simulink model "Transformer_Operating_Model"  (R2025b)
settings: Solver=ode23t  StartTime=0.0  StopTime=t_stop  MaxStep=t_step_max  RelTol=solver_reltol
PreLoadFcn:
  | if exist('params_transformer','file')~=2, addpath(fileparts(get_param(bdroot,'FileName'))); end; params_transformer;
InitFcn:
  | if exist('params_transformer','file')~=2, addpath(fileparts(get_param(bdroot,'FileName'))); end; params_transformer;
values from neighbouring files (symbols this model uses):
  dT_double_age = 6    [params_transformer.m]
  dTheta_hr = H_hs * g_r    (= 22.1)    [params_transformer.m]
  I_LV_rated = S_rated/(sqrt(3)*V_LV)    [params_transformer.m]
  k21 = 2    [params_transformer.m]
  P0 = 18e3    (= 18000)    [params_transformer.m]
  P_load_min = 1e-3*S_rated    (= 40000)    [params_transformer.m]
  P_tot_r = P0 + Pk    (= 154000)    [params_transformer.m]
  Pk = ukr_pct/100 * S_rated    (= 136000)    [params_transformer.m]
  R_th_h = 1    [params_transformer.m]
  S_rated = 40e6    (= 40000000)    [params_transformer.m]
  t_event_s = 60    [params_transformer.m]
  t_sample_s = t_sample_h*3600    [params_transformer.m]
  T_zero_C_in_K = 273.15    [params_transformer.m]
  theta_amb_C = 20    [params_transformer.m]    (also in run_step36.m = evalin('base', 'theta_amb_C'))
  theta_ref_age = 98    [params_transformer.m]
  x_oil = 0.8    [params_transformer.m]
  y_wdg = 1.3    [params_transformer.m]
libraries: fl_lib x16, nesl_utility x10, ee_lib x4, simulink x1
Description:
  | Transformer operating model (40 MVA, 110/20 kV): electrical network, losses, thermal network and ageing. Operating context only: no gas value is generated. Parameters: params_transformer.m. Built by build_Transformer_Operating_Model.m (MPhil project, Roadmap Step 33).
settings Model: Creator=Silas Asare  LastModifiedBy=Silas Asare
settings DebuggingCC: SignalInfNanChecking=error  UnconnectedInputMsg=error  UnconnectedOutputMsg=error  UnconnectedLineMsg=error  UniqueDataStoreMsg=error  StrictBusMsg=ErrorOnBusTreatedAsVector

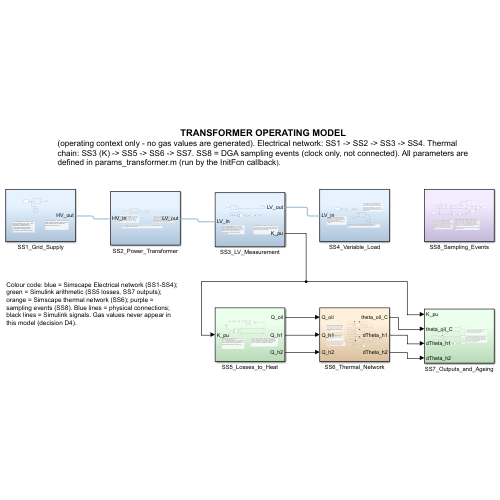
[thumbnail: Simulink's stored preview of the top-level diagram]
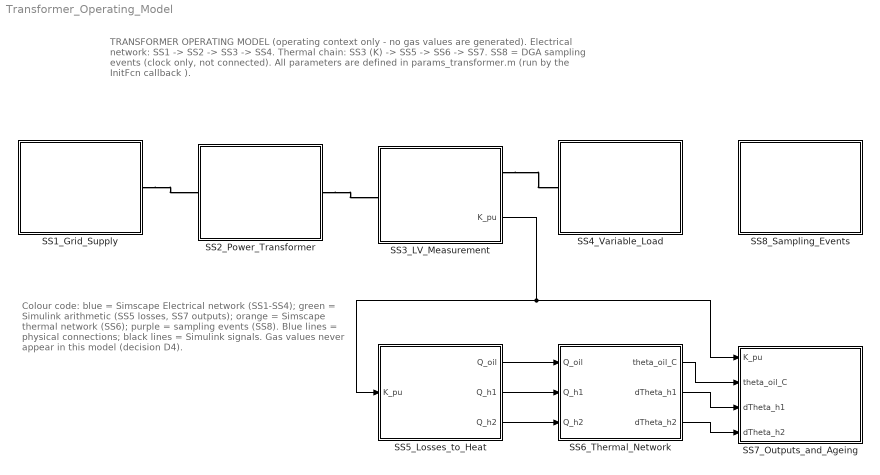
== system Transformer_Operating_Model ==
  note: TRANSFORMER OPERATING MODEL
      | (operating context only - no gas values are generated). Electrical network: SS1 -> SS2 -> SS3 -> SS4. Thermal chain: SS3 (K) -> SS5 -> SS6 -> SS7. SS8 = DGA sampling events (clock only, not connected). All parameters are defined in params_transformer.m (run by the InitFcn callback ).
  note: Colour code: blue = Simscape Electrical network (SS1-SS4); green = Simulink arithmetic (SS5 losses, SS7 outputs); orange = Simscape thermal network (SS6); purple = sampling events (SS8). Blue lines = physical connections; black lines = Simulink signals. Gas values never appear in this model (decision D4).
  SS1_Grid_Supply : Subsystem  Description=Simscape Electrical. Ideal 110 kV, 50 Hz three-phase source (infinite bus). Output HV_out.
  SS2_Power_Transformer : Subsystem  Description=Simscape Electrical. 40 MVA Delta/grounded-Wye transformer with winding resistance, leakage and magnetising branch. HV_in -> LV_out.
  SS3_LV_Measurement : Subsystem  Description=Simscape Electrical sensor + Simulink arithmetic. Measures the LV currents and outputs the load factor K_pu. LV_in -> LV_out, K_pu.
      settings: PortSchema="{\"entries\":[{\"content\":{\"sides\":[{\"content\":{\"connectorIds\":[\"LConn1\"]},\"type\":\"ConnectorPlacement.EquallySpacedRectSide\",\"uuid\":\"625cf4c8-f538-443e-9be6-835b81de7975\"},{\"content\":{\"connectorIds\":[\"RConn1\",\"Out1\"],\"side\":\"RIGHT\"},\"type\":\"ConnectorPlacement.EquallySpacedRectSide\",\"uuid\":\"310d5747-96d2-486e-a648-53e939d57def\"},{\"content\":{\"side\":\"TOP\"},\"type\":\"ConnectorPlacement.EquallySpacedRectSide\",\"uuid\":\"30abf6b0-d060-4f16-93ae-5727792815bb\"}]},\"type\":\"ConnectorPlacement.EquallySpacedConnector\",\"uuid\":\"dfd1b5c5-28ca-4eef-9e4a-4f0f0934eb6f\"}],\"packageUris\":[\"http://schema.mathworks.com/mf0/Connector/R2020b\"],\"version\":\"1.0\"}"
  SS4_Variable_Load : Subsystem  Description=Simscape Electrical + Simulink. Resistive three-phase load, P = K(t)*S_rated, from load_profile. Input LV_in.
  SS5_Losses_to_Heat : Subsystem  Description=Simulink. Heat inputs Q_oil, Q_h1, Q_h2 [W] from K_pu (IEC 60076-7 differential-equation model).
  SS6_Thermal_Network : Subsystem  Description=Simscape Foundation thermal. Three R-C circuits: top oil, hot-spot rise 1 and 2. Own Solver Configuration.
  SS7_Outputs_and_Ageing : Subsystem  Description=Simulink. Hot-spot temperature, relative ageing rate, and logging of K_pu, theta_oil_C, theta_hs_C, ageing_rate_V.
  SS8_Sampling_Events : Subsystem  Description=Simulink. DGA sampling events (Step 37): from the clock and t_sample_s it outputs record_index (row in heldout_record_ids) and sampling_event. Never a gas value; not connected to SS1-SS7.
  wires:
  SS3_LV_Measurement/1(K_pu) -> SS5_Losses_to_Heat/1(K_pu), SS7_Outputs_and_Ageing/1(K_pu)
  SS5_Losses_to_Heat/1(Q_oil) -> SS6_Thermal_Network/1(Q_oil)
  SS6_Thermal_Network/1(theta_oil_C) -> SS7_Outputs_and_Ageing/2(theta_oil_C)
  SS5_Losses_to_Heat/2(Q_h1) -> SS6_Thermal_Network/2(Q_h1)
  SS6_Thermal_Network/2(dTheta_h1) -> SS7_Outputs_and_Ageing/3(dTheta_h1)
  SS5_Losses_to_Heat/3(Q_h2) -> SS6_Thermal_Network/3(Q_h2)
  SS6_Thermal_Network/3(dTheta_h2) -> SS7_Outputs_and_Ageing/4(dTheta_h2)
  connections:
  SS1_Grid_Supply/RConn1 -- SS2_Power_Transformer/LConn1
  SS2_Power_Transformer/RConn1 -- SS3_LV_Measurement/LConn1
  SS3_LV_Measurement/RConn1 -- SS4_Variable_Load/LConn1

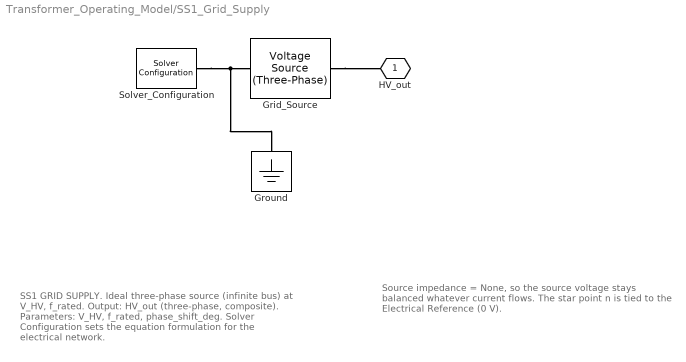
== system Transformer_Operating_Model/SS1_Grid_Supply ==
  note: SS1 GRID SUPPLY. Ideal three-phase source (infinite bus) at V_HV, f_rated. Output: HV_out (three-phase, composite). Parameters: V_HV, f_rated, phase_shift_deg. Solver Configuration sets the equation formulation for the electrical network.
  note: Source impedance = None, so the source voltage stays balanced whatever current flows. The star point n is tied to the Electrical Reference (0 V).
  Grid_Source : ee_lib/Sources/Voltage Source (Three-Phase)  vline_rms=V_HV V  shift=phase_shift_deg deg  freq=f_rated Hz  impedance_option=0  SShortCircuit=1e6 A*V  XR=15  R=0.01 Ohm  L=3.97e-4 H  harmonic_option=0  harmonic_orders=[5, 7, 11, 13]  harmonic_ratios=[.1, .1, .1, .1]  G_parasitic=0 1/Ohm  I_specify=off  I_priority=None  I=[0, 0, 0] A  I_nominal_specify=off  I_nominal_value=1  I_nominal_unit=A
  Ground : fl_lib/Electrical/Electrical Elements/Electrical Reference
  Solver_Configuration : nesl_utility/Solver Configuration  PhysicalDomain=network_engine_domain  SubClassName=solver  LeftPortType=input  RightPortType=generic  Tones=[]  Harmonics=[]  SimulateNoise=off  Profile=off  UseLocalSampling=off  EnableSwitchedLinearOptims=on  FrequencyDomain=off  UseCCode=off  RelTol=0.001  AbsTol=0.001  MinStep=1e-09  ToWorkspace=off  RevertToSquareIcSolve=off  NumHomotopyIterations=100  PhasorMode=off  PhasorModeNumHarmonics=1  ConsistencySolver=NEWTON_XTOL_AFTER_FTOL  IndexReductionMethod=DerivativeReplacement  DoDC=off  ResidualTolerance=1e-09  ConsistencyTolSource=GLOBAL  ConsistencyAbsTol=0.001  ConsistencyRelTol=0.001  ConsistencyTolFactor=0.001  UseLocalSolver=off  LocalSolverChoice=NE_BACKWARD_EULER_ADVANCER  ResolveIndetEquations=on  FunctionEvalNumThread=1  LocalSolverSampleTime=0.001  DoFixedCost=off  MaxNonlinIter=3  MaxModeIter=2  ComputeImpulses=off  ImpulseIterations=2  LinearAlgebra=auto  LinearAlgebraNumThread=0  EquationFormulation=NE_FREQUENCY_TIME_EF  DelaysMemoryBudget=1024  AutomaticFiltering=on  FilteringTimeConstant=0.001  PartitionStorageMethod=AS_NEEDED  PartitionMemoryBudget=1024  PartitionMethod=ROBUST  MultibodyUseLocalSolver=off  MultibodyLocalSolverChoice=ODE1  MultibodyLocalSolverSampleTime=0.001
  HV_out : PMIOPort  Side=Right
  connections:
  Grid_Source/RConn1 -- HV_out/RConn1
  Solver_Configuration/RConn1 -- Ground/LConn1 -- Grid_Source/LConn1

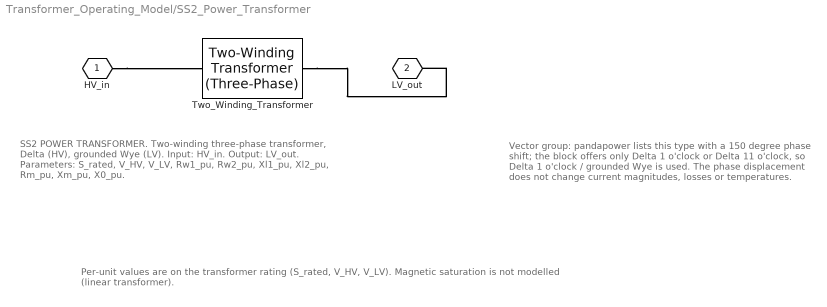
== system Transformer_Operating_Model/SS2_Power_Transformer ==
  note: SS2 POWER TRANSFORMER. Two-winding three-phase transformer, Delta (HV), grounded Wye (LV). Input: HV_in. Output: LV_out. Parameters: S_rated, V_HV, V_LV, Rw1_pu, Rw2_pu, Xl1_pu, Xl2_pu, Rm_pu, Xm_pu, X0_pu.
  note: Vector group: pandapower lists this type with a 150 degree phase shift; the block offers only Delta 1 o'clock or Delta 11 o'clock, so Delta 1 o'clock / grounded Wye is used. The phase displacement does not change current magnitudes, losses or temperatures.
  note: Per-unit values are on the transformer rating (S_rated, V_HV, V_LV). Magnetic saturation is not modelled (linear transformer).
  Two_Winding_Transformer : ee_lib/Passive/Transformers/Two-Winding Transformer (Three-Phase)  SRated=S_rated V*A  FRated=f_rated Hz  Winding1Connection=ee.enum.windingconnection.delta1  VRated1=V_HV V  Winding2Connection=ee.enum.windingconnection.Yg  VRated2=V_LV V  CoreType=ee.enum.coretype.threelimb  pu_Rw1=Rw1_pu  pu_Rw2=Rw2_pu  leakage_reactance_option=ee.enum.transformer_leakage.include  pu_Xl1=Xl1_pu  pu_Xl2=Xl2_pu  magnetizing_resistance_option=ee.enum.transformer_magnetizingResistance.include  pu_Rm=Rm_pu  magnetizing_reactance_option=ee.enum.transformer_magnetizingReactance.include  saturation_option=ee.enum.transformer_saturation.exclude  pu_Xm=Xm_pu  current_data=[0, .002, 1, 2]  magnetic_flux_data=[0, 1.2, 1.5, 1.51]  pu_X0=X0_pu  i1_specify=off  i1_priority=None  i1=[0, 0, 0] A  i1_nominal_specify=off  i1_nominal_value=1  i1_nominal_unit=A  i2_specify=off  i2_priority=None  i2=[0, 0, 0] A  i2_nominal_specify=off  i2_nominal_value=1  i2_nominal_unit=A  phi_specify=off  phi_priority=None  phi=[0, 0, 0]  phi_nominal_specify=off  phi_nominal_value=1  phi_nominal_unit=1  power_dissipated_specify=off  power_dissipated_priority=None  power_dissipated=0 W  power_dissipated_nominal_specify=off  power_dissipated_nominal_value=1  power_dissipated_nominal_unit=W
      settings: InternalSimscapePortConfiguration="{\"Bottom\":[],\"Left\":[{\"id\":\"N1\",\"label\":\"~1\",\"type\":\"foundation.electrical.three_phase\"}],\"Right\":[{\"id\":\"N2\",\"label\":\"~2\",\"type\":\"foundation.electrical.three_phase\"}],\"Top\":[]}"
  HV_in : PMIOPort  Side=Left
  LV_out : PMIOPort  Port=2  Side=Right
  connections:
  HV_in/RConn1 -- Two_Winding_Transformer/LConn1
  Two_Winding_Transformer/RConn1 -- LV_out/RConn1

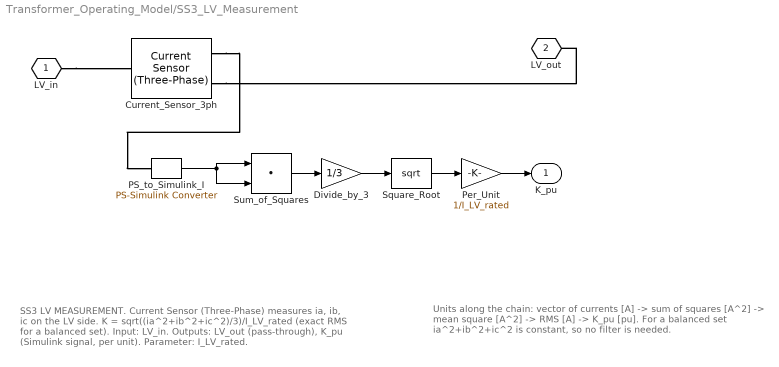
== system Transformer_Operating_Model/SS3_LV_Measurement ==
  note: SS3 LV MEASUREMENT. Current Sensor (Three-Phase) measures ia, ib, ic on the LV side. K = sqrt((ia^2+ib^2+ic^2)/3)/I_LV_rated (exact RMS for a balanced set). Input: LV_in. Outputs: LV_out (pass-through), K_pu (Simulink signal, per unit). Parameter: I_LV_rated.
  note: Units along the chain: vector of currents [A] -> sum of squares [A^2] -> mean square [A^2] -> RMS [A] -> K_pu [pu]. For a balanced set ia^2+ib^2+ic^2 is constant, so no filter is needed.
  Current_Sensor_3ph : ee_lib/Sensors & Transducers/Current Sensor (Three-Phase)
  Divide_by_3 : Gain  Gain=1/3
  PS_to_Simulink_I : nesl_utility/PS-Simulink Converter  PhysicalDomain=network_engine_domain  SubClassName=ps_output  LeftPortType=input  RightPortType=output  PseudoPeriodic=off  Frequencies=[]  VectorFormat=inherit  Unit=A  AffineConversion=off
  Per_Unit : Gain  Gain=1/I_LV_rated
  Square_Root : Sqrt
  Sum_of_Squares : DotProduct  OutDataTypeStr=Inherit: Inherit via internal rule
  LV_in : PMIOPort  Side=Left
  LV_out : PMIOPort  Port=2  Side=Right
  K_pu : Outport
  wires:
  PS_to_Simulink_I/1 -> Sum_of_Squares/1, Sum_of_Squares/2
  Sum_of_Squares/1 -> Divide_by_3/1
  Divide_by_3/1 -> Square_Root/1
  Square_Root/1 -> Per_Unit/1
  Per_Unit/1 -> K_pu/1
  connections:
  LV_in/RConn1 -- Current_Sensor_3ph/LConn1
  Current_Sensor_3ph/RConn2 -- LV_out/RConn1
  Current_Sensor_3ph/RConn1 -- PS_to_Simulink_I/LConn1

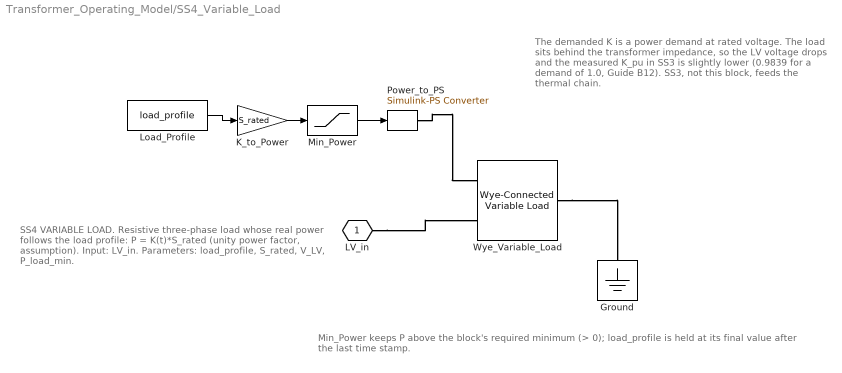
== system Transformer_Operating_Model/SS4_Variable_Load ==
  note: SS4 VARIABLE LOAD. Resistive three-phase load whose real power follows the load profile: P = K(t)*S_rated (unity power factor, assumption). Input: LV_in. Parameters: load_profile, S_rated, V_LV, P_load_min.
  note: The demanded K is a power demand at rated voltage. The load sits behind the transformer impedance, so the LV voltage drops and the measured K_pu in SS3 is slightly lower (0.9839 for a demand of 1.0, Guide B12). SS3, not this block, feeds the thermal chain.
  note: Min_Power keeps P above the block's required minimum (> 0); load_profile is held at its final value after the last time stamp.
  Ground : fl_lib/Electrical/Electrical Elements/Electrical Reference
  K_to_Power : Gain  Gain=S_rated
  Load_Profile : FromWorkspace  VariableName=load_profile  OutputAfterFinalValue=Holding final value
  Min_Power : Saturate  UpperLimit=inf  LowerLimit=P_load_min
  Power_to_PS : nesl_utility/Simulink-PS Converter  PhysicalDomain=network_engine_domain  SubClassName=ps_input  LeftPortType=input  RightPortType=output  PseudoPeriodic=off  Frequencies=[]  NoiseDistribution=none  NoiseParameters=[]  Unit=W  AffineConversion=off  FilteringAndDerivatives=provide  SimscapeFilterOrder=1  InputFilterTimeConstant=0.001  UdotUserProvided=0
  Wye_Variable_Load : ee_lib/Passive/RLC Assemblies/Wye-Connected Variable Load  VRated=V_LV V  Pmin=P_load_min W
      settings: InternalSimscapePortConfiguration="{\"Bottom\":[],\"Left\":[{\"id\":\"P\",\"label\":\"P\",\"type\":\"input\"},{\"id\":\"N\",\"label\":\"~\",\"type\":\"foundation.electrical.three_phase\"}],\"Right\":[{\"id\":\"n\",\"label\":\"n\",\"type\":\"foundation.electrical.electrical\"}],\"Top\":[]}"
  LV_in : PMIOPort  Side=Left
  wires:
  Load_Profile/1 -> K_to_Power/1
  K_to_Power/1 -> Min_Power/1
  Min_Power/1 -> Power_to_PS/1
  connections:
  LV_in/RConn1 -- Wye_Variable_Load/LConn2
  Wye_Variable_Load/RConn1 -- Ground/LConn1
  Power_to_PS/RConn1 -- Wye_Variable_Load/LConn1

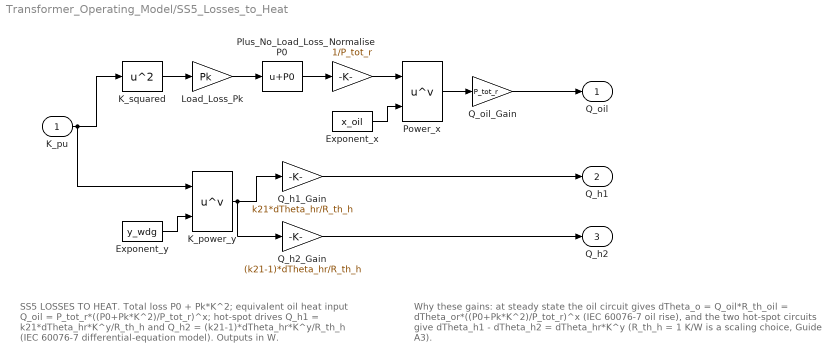
== system Transformer_Operating_Model/SS5_Losses_to_Heat ==
  note: SS5 LOSSES TO HEAT. Total loss P0 + Pk*K^2; equivalent oil heat input Q_oil = P_tot_r*((P0+Pk*K^2)/P_tot_r)^x; hot-spot drives Q_h1 = k21*dTheta_hr*K^y/R_th_h and Q_h2 = (k21-1)*dTheta_hr*K^y/R_th_h (IEC 60076-7 differential-equation model). Outputs in W.
  note: Why these gains: at steady state the oil circuit gives dTheta_o = Q_oil*R_th_oil = dTheta_or*((P0+Pk*K^2)/P_tot_r)^x (IEC 60076-7 oil rise), and the two hot-spot circuits give dTheta_h1 - dTheta_h2 = dTheta_hr*K^y (R_th_h = 1 K/W is a scaling choice, Guide A3).
  K_pu : Inport
  Exponent_x : Constant  Value=x_oil
  Exponent_y : Constant  Value=y_wdg
  K_power_y : Math  Operator=pow
  K_squared : Math  Operator=square
  Load_Loss_Pk : Gain  Gain=Pk
  Normalise : Gain  Gain=1/P_tot_r
  Plus_No_Load_Loss_P0 : Bias  Bias=P0  SaturateOnIntegerOverflow=off
  Power_x : Math  Operator=pow
  Q_h1_Gain : Gain  Gain=k21*dTheta_hr/R_th_h
  Q_h2_Gain : Gain  Gain=(k21-1)*dTheta_hr/R_th_h
  Q_oil_Gain : Gain  Gain=P_tot_r
  Q_oil : Outport
  Q_h1 : Outport  Port=2
  Q_h2 : Outport  Port=3
  wires:
  K_pu/1 -> K_squared/1, K_power_y/1
  K_squared/1 -> Load_Loss_Pk/1
  Load_Loss_Pk/1 -> Plus_No_Load_Loss_P0/1
  Plus_No_Load_Loss_P0/1 -> Normalise/1
  Normalise/1 -> Power_x/1
  Exponent_x/1 -> Power_x/2
  Power_x/1 -> Q_oil_Gain/1
  Q_oil_Gain/1 -> Q_oil/1
  Exponent_y/1 -> K_power_y/2
  K_power_y/1 -> Q_h1_Gain/1, Q_h2_Gain/1
  Q_h1_Gain/1 -> Q_h1/1
  Q_h2_Gain/1 -> Q_h2/1

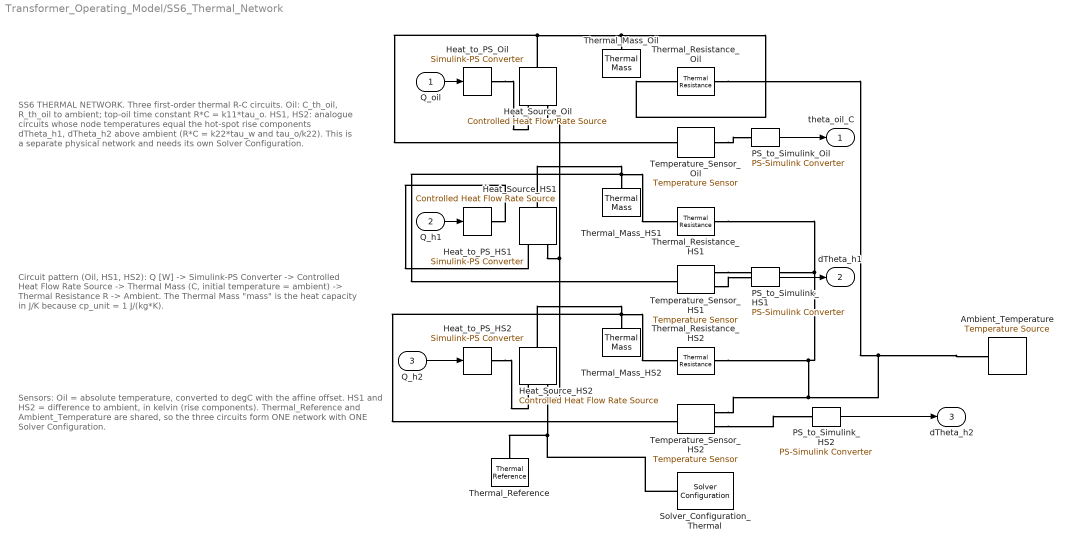
== system Transformer_Operating_Model/SS6_Thermal_Network ==
  note: SS6 THERMAL NETWORK. Three first-order thermal R-C circuits. Oil: C_th_oil, R_th_oil to ambient; top-oil time constant R*C = k11*tau_o. HS1, HS2: analogue circuits whose node temperatures equal the hot-spot rise components dTheta_h1, dTheta_h2 above ambient (R*C = k22*tau_w and tau_o/k22). This is a separate physical network and needs its own Solver Configuration.
  note: Circuit pattern (Oil, HS1, HS2): Q [W] -> Simulink-PS Converter -> Controlled Heat Flow Rate Source -> Thermal Mass (C, initial temperature = ambient) -> Thermal Resistance R -> Ambient. The Thermal Mass "mass" is the heat capacity in J/K because cp_unit = 1 J/(kg*K).
  note: Sensors: Oil = absolute temperature, converted to degC with the affine offset. HS1 and HS2 = difference to ambient, in kelvin (rise components). Thermal_Reference and Ambient_Temperature are shared, so the three circuits form ONE network with ONE Solver Configuration.
  Q_oil : Inport
  Q_h1 : Inport  Port=2
  Q_h2 : Inport  Port=3
  Ambient_Temperature : fl_lib/Thermal/Thermal Sources/Temperature Source  temperature=theta_amb_C + T_zero_C_in_K K
  Heat_Source_HS1 : fl_lib/Thermal/Thermal Sources/Controlled Heat Flow Rate Source
  Heat_Source_HS2 : fl_lib/Thermal/Thermal Sources/Controlled Heat Flow Rate Source
  Heat_Source_Oil : fl_lib/Thermal/Thermal Sources/Controlled Heat Flow Rate Source
  Heat_to_PS_HS1 : nesl_utility/Simulink-PS Converter  PhysicalDomain=network_engine_domain  SubClassName=ps_input  LeftPortType=input  RightPortType=output  PseudoPeriodic=off  Frequencies=[]  NoiseDistribution=none  NoiseParameters=[]  Unit=W  AffineConversion=off  FilteringAndDerivatives=provide  SimscapeFilterOrder=1  InputFilterTimeConstant=0.001  UdotUserProvided=0
  Heat_to_PS_HS2 : nesl_utility/Simulink-PS Converter  PhysicalDomain=network_engine_domain  SubClassName=ps_input  LeftPortType=input  RightPortType=output  PseudoPeriodic=off  Frequencies=[]  NoiseDistribution=none  NoiseParameters=[]  Unit=W  AffineConversion=off  FilteringAndDerivatives=provide  SimscapeFilterOrder=1  InputFilterTimeConstant=0.001  UdotUserProvided=0
  Heat_to_PS_Oil : nesl_utility/Simulink-PS Converter  PhysicalDomain=network_engine_domain  SubClassName=ps_input  LeftPortType=input  RightPortType=output  PseudoPeriodic=off  Frequencies=[]  NoiseDistribution=none  NoiseParameters=[]  Unit=W  AffineConversion=off  FilteringAndDerivatives=provide  SimscapeFilterOrder=1  InputFilterTimeConstant=0.001  UdotUserProvided=0
  PS_to_Simulink_HS1 : nesl_utility/PS-Simulink Converter  PhysicalDomain=network_engine_domain  SubClassName=ps_output  LeftPortType=input  RightPortType=output  PseudoPeriodic=off  Frequencies=[]  VectorFormat=inherit  Unit=K  AffineConversion=off
  PS_to_Simulink_HS2 : nesl_utility/PS-Simulink Converter  PhysicalDomain=network_engine_domain  SubClassName=ps_output  LeftPortType=input  RightPortType=output  PseudoPeriodic=off  Frequencies=[]  VectorFormat=inherit  Unit=K  AffineConversion=off
  PS_to_Simulink_Oil : nesl_utility/PS-Simulink Converter  PhysicalDomain=network_engine_domain  SubClassName=ps_output  LeftPortType=input  RightPortType=output  PseudoPeriodic=off  Frequencies=[]  VectorFormat=inherit  Unit=degC  AffineConversion=on
  Solver_Configuration_Thermal : nesl_utility/Solver Configuration  PhysicalDomain=network_engine_domain  SubClassName=solver  LeftPortType=input  RightPortType=generic  Tones=[]  Harmonics=[]  SimulateNoise=off  Profile=off  UseLocalSampling=off  EnableSwitchedLinearOptims=on  FrequencyDomain=off  UseCCode=off  RelTol=0.001  AbsTol=0.001  MinStep=1e-09  ToWorkspace=off  RevertToSquareIcSolve=off  NumHomotopyIterations=100  PhasorMode=off  PhasorModeNumHarmonics=1  ConsistencySolver=NEWTON_XTOL_AFTER_FTOL  IndexReductionMethod=DerivativeReplacement  DoDC=off  ResidualTolerance=1e-09  ConsistencyTolSource=GLOBAL  ConsistencyAbsTol=0.001  ConsistencyRelTol=0.001  ConsistencyTolFactor=0.001  UseLocalSolver=off  LocalSolverChoice=NE_BACKWARD_EULER_ADVANCER  ResolveIndetEquations=on  FunctionEvalNumThread=1  LocalSolverSampleTime=0.001  DoFixedCost=off  MaxNonlinIter=3  MaxModeIter=2  ComputeImpulses=off  ImpulseIterations=2  LinearAlgebra=auto  LinearAlgebraNumThread=0  EquationFormulation=NE_TIME_EF  DelaysMemoryBudget=1024  AutomaticFiltering=on  FilteringTimeConstant=0.001  PartitionStorageMethod=AS_NEEDED  PartitionMemoryBudget=1024  PartitionMethod=ROBUST  MultibodyUseLocalSolver=off  MultibodyLocalSolverChoice=ODE1  MultibodyLocalSolverSampleTime=0.001
  Temperature_Sensor_HS1 : fl_lib/Thermal/Thermal Sensors/Temperature Sensor  temperature_measure=foundation.enum.MeasurementReference.difference
  Temperature_Sensor_HS2 : fl_lib/Thermal/Thermal Sensors/Temperature Sensor  temperature_measure=foundation.enum.MeasurementReference.difference
  Temperature_Sensor_Oil : fl_lib/Thermal/Thermal Sensors/Temperature Sensor  temperature_measure=foundation.enum.MeasurementReference.absolute
      settings: InternalSimscapePortConfiguration="{\"Bottom\":[],\"Left\":[{\"id\":\"A\",\"label\":\"A\",\"type\":\"foundation.thermal.thermal\"}],\"Right\":[{\"id\":\"T\",\"label\":\"T\",\"type\":\"output\"}],\"Top\":[]}"
  Thermal_Mass_HS1 : fl_lib/Thermal/Thermal Elements/Thermal Mass  mass_type=foundation.enum.constant_variable.constant  mass=C_th_h1 kg  sp_heat=cp_unit J/(kg*K)  mass_min=1e-6 kg  num_ports=foundation.enum.numPorts2.one  m_specify=off  m_priority=High  m=1 kg  m_nominal_specify=off  m_nominal_value=1  m_nominal_unit=kg  T_specify=on  T_priority=High  T=theta_amb_C + T_zero_C_in_K K  T_nominal_specify=off  T_nominal_value=1  T_nominal_unit=K  Q_specify=off  Q_priority=None  Q=0 W  Q_nominal_specify=off  Q_nominal_value=1  Q_nominal_unit=W
  Thermal_Mass_HS2 : fl_lib/Thermal/Thermal Elements/Thermal Mass  mass_type=foundation.enum.constant_variable.constant  mass=C_th_h2 kg  sp_heat=cp_unit J/(kg*K)  mass_min=1e-6 kg  num_ports=foundation.enum.numPorts2.one  m_specify=off  m_priority=High  m=1 kg  m_nominal_specify=off  m_nominal_value=1  m_nominal_unit=kg  T_specify=on  T_priority=High  T=theta_amb_C + T_zero_C_in_K K  T_nominal_specify=off  T_nominal_value=1  T_nominal_unit=K  Q_specify=off  Q_priority=None  Q=0 W  Q_nominal_specify=off  Q_nominal_value=1  Q_nominal_unit=W
  Thermal_Mass_Oil : fl_lib/Thermal/Thermal Elements/Thermal Mass  mass_type=foundation.enum.constant_variable.constant  mass=C_th_oil kg  sp_heat=cp_unit J/(kg*K)  mass_min=1e-6 kg  num_ports=foundation.enum.numPorts2.one  m_specify=off  m_priority=High  m=1 kg  m_nominal_specify=off  m_nominal_value=1  m_nominal_unit=kg  T_specify=on  T_priority=High  T=theta_amb_C + T_zero_C_in_K K  T_nominal_specify=off  T_nominal_value=1  T_nominal_unit=K  Q_specify=off  Q_priority=None  Q=0 W  Q_nominal_specify=off  Q_nominal_value=1  Q_nominal_unit=W
  Thermal_Reference : fl_lib/Thermal/Thermal Elements/Thermal Reference
  Thermal_Resistance_HS1 : fl_lib/Thermal/Thermal Elements/Thermal Resistance  resistance=R_th_h K/W  T_specify=off  T_priority=None  T=0 K  T_nominal_specify=off  T_nominal_value=1  T_nominal_unit=K  Q_specify=off  Q_priority=None  Q=0 W  Q_nominal_specify=off  Q_nominal_value=1  Q_nominal_unit=W
  Thermal_Resistance_HS2 : fl_lib/Thermal/Thermal Elements/Thermal Resistance  resistance=R_th_h K/W  T_specify=off  T_priority=None  T=0 K  T_nominal_specify=off  T_nominal_value=1  T_nominal_unit=K  Q_specify=off  Q_priority=None  Q=0 W  Q_nominal_specify=off  Q_nominal_value=1  Q_nominal_unit=W
  Thermal_Resistance_Oil : fl_lib/Thermal/Thermal Elements/Thermal Resistance  resistance=R_th_oil K/W  T_specify=off  T_priority=None  T=0 K  T_nominal_specify=off  T_nominal_value=1  T_nominal_unit=K  Q_specify=off  Q_priority=None  Q=0 W  Q_nominal_specify=off  Q_nominal_value=1  Q_nominal_unit=W
  theta_oil_C : Outport
  dTheta_h1 : Outport  Port=2
  dTheta_h2 : Outport  Port=3
  wires:
  Q_oil/1 -> Heat_to_PS_Oil/1
  PS_to_Simulink_Oil/1 -> theta_oil_C/1
  Q_h1/1 -> Heat_to_PS_HS1/1
  PS_to_Simulink_HS1/1 -> dTheta_h1/1
  Q_h2/1 -> Heat_to_PS_HS2/1
  PS_to_Simulink_HS2/1 -> dTheta_h2/1
  connections:
  Heat_to_PS_Oil/RConn1 -- Heat_Source_Oil/RConn1
  Heat_Source_Oil/RConn2 -- Heat_Source_HS1/RConn2 -- Thermal_Reference/LConn1 -- Solver_Configuration_Thermal/RConn1 -- Heat_Source_HS2/RConn2
  Heat_Source_Oil/LConn1 -- Thermal_Mass_Oil/LConn1 -- Thermal_Resistance_Oil/LConn1 -- Temperature_Sensor_Oil/LConn1
  Thermal_Resistance_Oil/RConn1 -- Temperature_Sensor_HS1/RConn1 -- Thermal_Resistance_HS1/RConn1 -- Thermal_Resistance_HS2/RConn1 -- Temperature_Sensor_HS2/RConn1 -- Ambient_Temperature/LConn1
  Temperature_Sensor_Oil/RConn1 -- PS_to_Simulink_Oil/LConn1
  Heat_to_PS_HS1/RConn1 -- Heat_Source_HS1/RConn1
  Heat_Source_HS1/LConn1 -- Thermal_Mass_HS1/LConn1 -- Temperature_Sensor_HS1/LConn1 -- Thermal_Resistance_HS1/LConn1
  Temperature_Sensor_HS1/RConn2 -- PS_to_Simulink_HS1/LConn1
  Heat_to_PS_HS2/RConn1 -- Heat_Source_HS2/RConn1
  Heat_Source_HS2/LConn1 -- Thermal_Mass_HS2/LConn1 -- Temperature_Sensor_HS2/LConn1 -- Thermal_Resistance_HS2/LConn1
  Temperature_Sensor_HS2/RConn2 -- PS_to_Simulink_HS2/LConn1

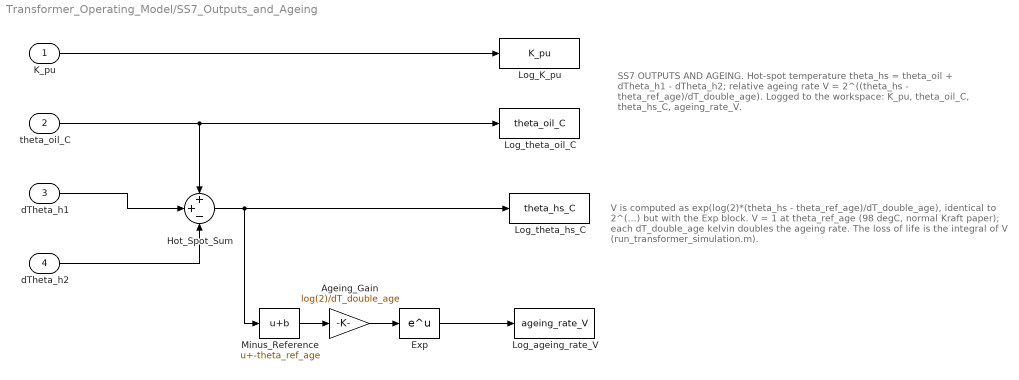
== system Transformer_Operating_Model/SS7_Outputs_and_Ageing ==
  note: SS7 OUTPUTS AND AGEING. Hot-spot temperature theta_hs = theta_oil + dTheta_h1 - dTheta_h2; relative ageing rate V = 2^((theta_hs - theta_ref_age)/dT_double_age). Logged to the workspace: K_pu, theta_oil_C, theta_hs_C, ageing_rate_V.
  note: V is computed as exp(log(2)*(theta_hs - theta_ref_age)/dT_double_age), identical to 2^(...) but with the Exp block. V = 1 at theta_ref_age (98 degC, normal Kraft paper); each dT_double_age kelvin doubles the ageing rate. The loss of life is the integral of V (run_transformer_simulation.m).
  K_pu : Inport
  theta_oil_C : Inport  Port=2
  dTheta_h1 : Inport  Port=3
  dTheta_h2 : Inport  Port=4
  Ageing_Gain : Gain  Gain=log(2)/dT_double_age
  Exp : Math
  Hot_Spot_Sum : Sum  Inputs=++-
  Log_K_pu : ToWorkspace  VariableName=K_pu  SaveFormat=Timeseries  SampleTime=-1
  Log_ageing_rate_V : ToWorkspace  VariableName=ageing_rate_V  SaveFormat=Timeseries  SampleTime=-1
  Log_theta_hs_C : ToWorkspace  VariableName=theta_hs_C  SaveFormat=Timeseries  SampleTime=-1
  Log_theta_oil_C : ToWorkspace  VariableName=theta_oil_C  SaveFormat=Timeseries  SampleTime=-1
  Minus_Reference : Bias  Bias=-theta_ref_age  SaturateOnIntegerOverflow=off
  wires:
  theta_oil_C/1 -> Log_theta_oil_C/1, Hot_Spot_Sum/1
  dTheta_h1/1 -> Hot_Spot_Sum/2
  dTheta_h2/1 -> Hot_Spot_Sum/3
  Hot_Spot_Sum/1 -> Minus_Reference/1, Log_theta_hs_C/1
  Minus_Reference/1 -> Ageing_Gain/1
  Ageing_Gain/1 -> Exp/1
  K_pu/1 -> Log_K_pu/1
  Exp/1 -> Log_ageing_rate_V/1

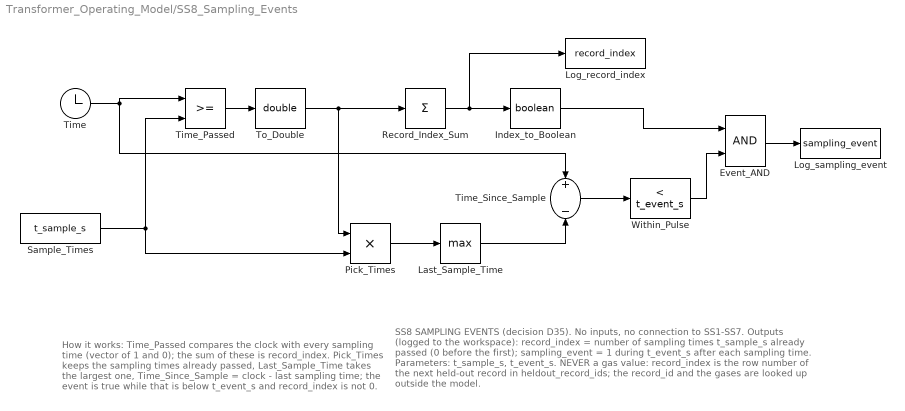
== system Transformer_Operating_Model/SS8_Sampling_Events ==
  note: SS8 SAMPLING EVENTS (decision D35). No inputs, no connection to SS1-SS7. Outputs (logged to the workspace): record_index = number of sampling times t_sample_s already passed (0 before the first); sampling_event = 1 during t_event_s after each sampling time. Parameters: t_sample_s, t_event_s. NEVER a gas value: record_index is the row number of the next held-out record in heldout_record_ids; the record_id and the gases are looked up outside the model.
  note: How it works: Time_Passed compares the clock with every sampling time (vector of 1 and 0); the sum of these is record_index. Pick_Times keeps the sampling times already passed, Last_Sample_Time takes the largest one, Time_Since_Sample = clock - last sampling time; the event is true while that is below t_event_s and record_index is not 0.
  Event_AND : Logic  AllPortsSameDT=off  OutDataTypeStr=boolean
  Index_to_Boolean : DataTypeConversion  OutDataTypeStr=boolean  SaturateOnIntegerOverflow=off  RndMeth=Floor
  Last_Sample_Time : MinMax  Function=max
  Log_record_index : ToWorkspace  VariableName=record_index  SaveFormat=Timeseries  SampleTime=-1
  Log_sampling_event : ToWorkspace  VariableName=sampling_event  SaveFormat=Timeseries  SampleTime=-1
  Pick_Times : Product  Inputs=**
  Record_Index_Sum : Sum  Inputs=+
  Sample_Times : Constant  Value=t_sample_s
  Time : Clock
  Time_Passed : RelationalOperator  OutDataTypeStr=boolean  RndMeth=Simplest  InputSameDT=off
  Time_Since_Sample : Sum  Inputs=+-
  To_Double : DataTypeConversion  OutDataTypeStr=double  SaturateOnIntegerOverflow=off  RndMeth=Floor
  Within_Pulse : simulink/Logic and Bit Operations/Compare To Constant  relop=<  const=t_event_s  OutDataTypeStr=boolean
  wires:
  Time/1 -> Time_Passed/1, Time_Since_Sample/1
  Sample_Times/1 -> Time_Passed/2, Pick_Times/2
  Time_Passed/1 -> To_Double/1
  To_Double/1 -> Record_Index_Sum/1, Pick_Times/1
  Pick_Times/1 -> Last_Sample_Time/1
  Last_Sample_Time/1 -> Time_Since_Sample/2
  Time_Since_Sample/1 -> Within_Pulse/1
  Record_Index_Sum/1 -> Log_record_index/1, Index_to_Boolean/1
  Within_Pulse/1 -> Event_AND/2
  Index_to_Boolean/1 -> Event_AND/1
  Event_AND/1 -> Log_sampling_event/1
